simulink model "nms_sim_2D_cost"  (R2024b)
settings: Solver=ode15s  StartTime=0.0  StopTime=t_sim  MaxStep=dt_max  EnableMultiTasking=on
values from neighbouring files (symbols this model uses):
  a_BFSH = param_ctrl(35)*1    [setCtrlPar_optim_CPGreflex2001_2D.m]
  a_GAS = param_ctrl(37)*1    [setCtrlPar_optim_CPGreflex2001_2D.m]
  a_GLU = param_ctrl(31)*1    [setCtrlPar_optim_CPGreflex2001_2D.m]
  a_HAM = param_ctrl(33)*1    [setCtrlPar_optim_CPGreflex2001_2D.m]
  a_HFL = param_ctrl(32)*1    [setCtrlPar_optim_CPGreflex2001_2D.m]
  a_RF = param_ctrl(34)*1    [setCtrlPar_optim_CPGreflex2001_2D.m]
  a_SOL = param_ctrl(38)*1    [setCtrlPar_optim_CPGreflex2001_2D.m]
  a_TA = param_ctrl(39)*1    [setCtrlPar_optim_CPGreflex2001_2D.m]
  a_VAS = param_ctrl(36)*1    [setCtrlPar_optim_CPGreflex2001_2D.m]
  ai = param_ctrl(96)*2.0    [setCtrlPar_optim_CPGreflex2001_2D.m]
  b_BFSH = param_ctrl(52)*.51    [setCtrlPar_optim_CPGreflex2001_2D.m]
  b_BFSHGAS = param_ctrl(55)*.51    [setCtrlPar_optim_CPGreflex2001_2D.m]
  b_BFSHHAM = param_ctrl(54)*.51    [setCtrlPar_optim_CPGreflex2001_2D.m]
  b_BFSHVAS = param_ctrl(53)*.51    [setCtrlPar_optim_CPGreflex2001_2D.m]
  b_GAS = param_ctrl(59)*.51    [setCtrlPar_optim_CPGreflex2001_2D.m]
  b_GASBFSH = param_ctrl(60)*.51    [setCtrlPar_optim_CPGreflex2001_2D.m]
  b_GASSOL = param_ctrl(61)*.51    [setCtrlPar_optim_CPGreflex2001_2D.m]
  b_GLU = param_ctrl(40)*.51    [setCtrlPar_optim_CPGreflex2001_2D.m]
  b_GLUHAM = param_ctrl(42)*.51    [setCtrlPar_optim_CPGreflex2001_2D.m]
  b_GLUHFL = param_ctrl(41)*.51    [setCtrlPar_optim_CPGreflex2001_2D.m]
  b_HAM = param_ctrl(46)*.51    [setCtrlPar_optim_CPGreflex2001_2D.m]
  b_HAMBFSH = param_ctrl(48)*.51    [setCtrlPar_optim_CPGreflex2001_2D.m]
  b_HAMGLU = param_ctrl(47)*.51    [setCtrlPar_optim_CPGreflex2001_2D.m]
  b_HFL = param_ctrl(43)*.51    [setCtrlPar_optim_CPGreflex2001_2D.m]
  b_HFLGLU = param_ctrl(44)*.51    [setCtrlPar_optim_CPGreflex2001_2D.m]
  b_HFLRF = param_ctrl(45)*.51    [setCtrlPar_optim_CPGreflex2001_2D.m]
  b_RF = param_ctrl(49)*.51    [setCtrlPar_optim_CPGreflex2001_2D.m]
  b_RFHFL = param_ctrl(50)*.51    [setCtrlPar_optim_CPGreflex2001_2D.m]
  b_RFVAS = param_ctrl(51)*.51    [setCtrlPar_optim_CPGreflex2001_2D.m]
  b_SOL = param_ctrl(62)*.51    [setCtrlPar_optim_CPGreflex2001_2D.m]
  b_SOLGAS = param_ctrl(64)*.51    [setCtrlPar_optim_CPGreflex2001_2D.m]
  b_SOLTA = param_ctrl(63)*.51    [setCtrlPar_optim_CPGreflex2001_2D.m]
  b_TA = param_ctrl(65)*.51    [setCtrlPar_optim_CPGreflex2001_2D.m]
  b_TASOL = param_ctrl(66)*.51    [setCtrlPar_optim_CPGreflex2001_2D.m]
  b_VAS = param_ctrl(56)*.51    [setCtrlPar_optim_CPGreflex2001_2D.m]
  b_VASBFSH = param_ctrl(57)*.51    [setCtrlPar_optim_CPGreflex2001_2D.m]
  b_VASRF = param_ctrl(58)*.51    [setCtrlPar_optim_CPGreflex2001_2D.m]
  bias = param_ctrl(97)*2.5    [setCtrlPar_optim_CPGreflex2001_2D.m]
  c = 0.05    [nms_MS_2D_scaled.m]
  c_jointstop = 0.3 / (pi/180)    (= 17.1887338539)    [nms_MS_2D_scaled.m]
  D12_F = 0.16    *scaleL_JPhys    [nms_MechInit_2D_scaleSkel.m]
  D12_S = 0.2460	*sub_height    [nms_MechInit_2D_scaleSkel.m]
  D12_T = 0.2450  *sub_height    [nms_MechInit_2D_scaleSkel.m]
  D12y_F = 0.039  *sub_height    [nms_MechInit_2D_scaleSkel.m]
  D12z_HAT = 0.1    [nms_MS_2D_scaled.m]
  D13_F = 0.20    *scaleL_JPhys    [nms_MechInit_2D_scaleSkel.m]
  D1G_F = 0.14    *scaleL_JPhys    [nms_MechInit_2D_scaleSkel.m]
  D1G_HAT = 0.35  *scaleL_JPhys    [nms_MechInit_2D_scaleSkel.m]
  D1G_S = (0.3 - D12y_F/4)	*scaleL_JPhys    [nms_MechInit_2D_scaleSkel.m]
  D1G_T = (0.3 - D12y_F/4)	*scaleL_JPhys    [nms_MechInit_2D_scaleSkel.m]
  D1Gy_F = D12y_F*D1G_F/D12_F    (= 0.07)    [nms_MechInit_2D_scaleSkel.m]
  d_BFSH = param_ctrl(26)*1    [setCtrlPar_optim_CPGreflex2001_2D.m]
  d_GAS = param_ctrl(28)*1    [setCtrlPar_optim_CPGreflex2001_2D.m]
  d_GLU = param_ctrl(22)*1    [setCtrlPar_optim_CPGreflex2001_2D.m]
  d_HAM = param_ctrl(24)*1    [setCtrlPar_optim_CPGreflex2001_2D.m]
  d_HFL = param_ctrl(23)*1    [setCtrlPar_optim_CPGreflex2001_2D.m]
  d_RF = param_ctrl(25)*1    [setCtrlPar_optim_CPGreflex2001_2D.m]
  d_SOL = param_ctrl(29)*1    [setCtrlPar_optim_CPGreflex2001_2D.m]
  d_TA = param_ctrl(30)*1    [setCtrlPar_optim_CPGreflex2001_2D.m]
  d_VAS = param_ctrl(27)*1    [setCtrlPar_optim_CPGreflex2001_2D.m]
  DeltaThRef = 5e-3    (= 0.005)    [nms_MS_2D_scaled.m]
  dloptBFSH = 3.0    (= 3)    [setCtrlPar_optim_CPGreflex2001_2D.m]
  dloptGAS = 3.0    (= 3)    [setCtrlPar_optim_CPGreflex2001_2D.m]
  dloptGLU = 3.0    (= 3)    [setCtrlPar_optim_CPGreflex2001_2D.m]
  dloptHAM = 3.0    (= 3)    [setCtrlPar_optim_CPGreflex2001_2D.m]
  dloptHFL = 3.0    (= 3)    [setCtrlPar_optim_CPGreflex2001_2D.m]
  dloptRF = 3.0    (= 3)    [setCtrlPar_optim_CPGreflex2001_2D.m]
  dloptSOL = 3.0    (= 3)    [setCtrlPar_optim_CPGreflex2001_2D.m]
  dloptTA = 3.0    (= 3)    [setCtrlPar_optim_CPGreflex2001_2D.m]
  dloptVAS = 3.0    (= 3)    [setCtrlPar_optim_CPGreflex2001_2D.m]
  ec_BFSH = param_ctrl(80)*0.15    [setCtrlPar_optim_CPGreflex2001_2D.m]
  ec_GAS = param_ctrl(82)*0.15    [setCtrlPar_optim_CPGreflex2001_2D.m]
  ec_GLU = param_ctrl(76)*0.15    [setCtrlPar_optim_CPGreflex2001_2D.m]
  ec_HAM = param_ctrl(78)*0.15    [setCtrlPar_optim_CPGreflex2001_2D.m]
  ec_HFL = param_ctrl(77)*0.15    [setCtrlPar_optim_CPGreflex2001_2D.m]
  ec_RF = param_ctrl(79)*0.15    [setCtrlPar_optim_CPGreflex2001_2D.m]
  ec_TA = param_ctrl(84)*0.15    [setCtrlPar_optim_CPGreflex2001_2D.m]
  ec_VAS = param_ctrl(81)*0.15    [setCtrlPar_optim_CPGreflex2001_2D.m]
  eref = 0.04    [nms_MS_2D_scaled.m]
  eref_GAS = 0.1    [nms_MS_2D_scaled.m]
  eref_SOL = 0.1    [nms_MS_2D_scaled.m]
  es_BFSH = param_ctrl(89)*0.15    [setCtrlPar_optim_CPGreflex2001_2D.m]
  es_GAS = param_ctrl(91)*0.15    [setCtrlPar_optim_CPGreflex2001_2D.m]
  es_GLU = param_ctrl(85)*0.15    [setCtrlPar_optim_CPGreflex2001_2D.m]
  es_HAM = param_ctrl(87)*0.15    [setCtrlPar_optim_CPGreflex2001_2D.m]
  es_HFL = param_ctrl(86)*0.15    [setCtrlPar_optim_CPGreflex2001_2D.m]
  es_RF = param_ctrl(88)*0.15    [setCtrlPar_optim_CPGreflex2001_2D.m]
  es_TA = param_ctrl(93)*0.15    [setCtrlPar_optim_CPGreflex2001_2D.m]
  es_VAS = param_ctrl(90)*0.15    [setCtrlPar_optim_CPGreflex2001_2D.m]
  FmaxBFSH = 350    [nms_MS_2D_scaled.m]
  FmaxGAS = 2000    [nms_MS_2D_scaled.m]
  FmaxGLU = 4000    [nms_MS_2D_scaled.m]
  FmaxHAM = 2000    [nms_MS_2D_scaled.m]
  FmaxHFL = 2000    [nms_MS_2D_scaled.m]
  FmaxRF = 850    [nms_MS_2D_scaled.m]
  FmaxSOL = 4000    [nms_MS_2D_scaled.m]
  FmaxTA = 800    [nms_MS_2D_scaled.m]
  FmaxVAS = 5000    [nms_MS_2D_scaled.m]
  g = 9.81    [nms_MS_2D_scaled.m]
  gamma_4 = param_ctrl(11) * 1.7    [setCtrlPar_optim_CPGreflexsynergy2023_2D.m]
  h_BFSH = param_ctrl(71)*.1    [setCtrlPar_optim_CPGreflex2001_2D.m]
  h_GAS = param_ctrl(73)*.1    [setCtrlPar_optim_CPGreflex2001_2D.m]
  h_GLU = param_ctrl(67)*.1    [setCtrlPar_optim_CPGreflex2001_2D.m]
  h_HAM = param_ctrl(69)*.1    [setCtrlPar_optim_CPGreflex2001_2D.m]
  h_HFL = param_ctrl(68)*.1    [setCtrlPar_optim_CPGreflex2001_2D.m]
  h_RF = param_ctrl(70)*.1    [setCtrlPar_optim_CPGreflex2001_2D.m]
  h_SOL = param_ctrl(74)*.1    [setCtrlPar_optim_CPGreflex2001_2D.m]
  h_TA = param_ctrl(75)*.1    [setCtrlPar_optim_CPGreflex2001_2D.m]
  h_VAS = param_ctrl(72)*.1    [setCtrlPar_optim_CPGreflex2001_2D.m]
  HLCtrlPar = [theta_tgt l_clr alpha_tgt alpha_cd alpha_cv]    [setCtrlPar_optim_reflex2015_2D.m]
  In_F = 0.005    *scaleM*scaleL_JPhys^2    [nms_MechInit_2D_scaleSkel.m]
  In_HAT = 2.5    *scaleM*scaleL_JPhys^2    [nms_MechInit_2D_scaleSkel.m]
  In_S = 0.05     *scaleM*scaleL_JPhys^2    [nms_MechInit_2D_scaleSkel.m]
  In_T = 0.15     *scaleM*scaleL_JPhys^2    [nms_MechInit_2D_scaleSkel.m]
  init_exc = 0.01    [setInitPar_optim_2D.m]
  init_fm = 0.01    [setInitPar_optim_2D.m]
  init_lce = 1    [setInitPar_optim_2D.m]
  init_LCPG = param_ctrl(12) * 0.01    [setCtrlPar_optim_CPGreflexsynergy2023_2D.m]
  init_LStance = 1    [setInitPar_optim_2D.m]
  init_N1 = osc_signal1(phi_off_osc_ind)    [setCtrlPar_optim_CPGreflex2001_2D.m]
  ... (+441 more)
undefined symbols (not defined in the file or in its folder): cost_act_exponent, cost_v_tgt, flag_controller, Newton, nStep_obj, nStep_startKin, Raphson, sgn, SSW_kin, terrain_slope_angle, v_plateS1, X, Y, Z
libraries: nesl_utility x94, sm_lib x90, simulink x28, simulink_extras x12
(part 13 of 20)

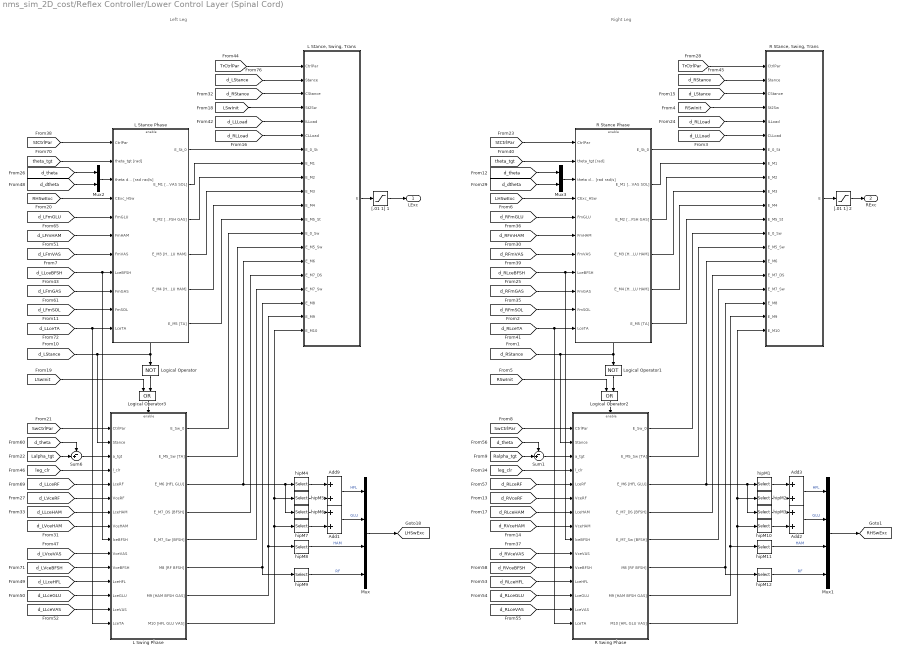
== system nms_sim_2D_cost/Reflex Controller/Lower Control Layer (Spinal Cord) ==
  note: Right Leg
  note: Left Leg
  Add{1..3,9} (4 alike) : Sum  Inputs=2
  L Stance Phase : Subsystem  TreatAsAtomicUnit=on
  "L Stance, Swing, Trans" : Subsystem
  L Swing Phase : Subsystem  TreatAsAtomicUnit=on
  Logical Operator : Logic  Operator=NOT  AllPortsSameDT=off  OutDataTypeStr=boolean
  Logical Operator1 : Logic  Operator=NOT  AllPortsSameDT=off  OutDataTypeStr=boolean
  Logical Operator2 : Logic  Operator=OR  AllPortsSameDT=off  OutDataTypeStr=boolean
  Logical Operator3 : Logic  Operator=OR  AllPortsSameDT=off  OutDataTypeStr=boolean
  Mux : Mux
  Mux1 : Mux
  Mux2 : Mux  Inputs=2
  Mux3 : Mux  Inputs=2
  R Stance Phase : Subsystem  TreatAsAtomicUnit=on
  "R Stance, Swing, Trans" : Subsystem
  R Swing Phase : Subsystem  TreatAsAtomicUnit=on
  Sum1 : Sum  Inputs=-+|
  Sum6 : Sum  Inputs=-+|
  "[.01 1] 1" : Saturate  UpperLimit=1  LowerLimit=0.01  ZeroCross=off
  "[.01 1] 2" : Saturate  UpperLimit=1  LowerLimit=0.01  ZeroCross=off
  hipM{1,4,9,12} (4 alike) : Selector  InputPortWidth=2  IndexOptions=Index vector (dialog)  Indices=1  OutputSizes=1
  hipM10 : Selector  InputPortWidth=3  IndexOptions=Index vector (dialog)  Indices=2  OutputSizes=1
  hipM{2,5,8,11} (4 alike) : Selector  InputPortWidth=3  IndexOptions=Index vector (dialog)  Indices=1  OutputSizes=1
  hipM3 : Selector  InputPortWidth=2  IndexOptions=Index vector (dialog)  Indices=2  OutputSizes=1
  hipM6 : Selector  InputPortWidth=2  IndexOptions=Index vector (dialog)  Indices=2  OutputSizes=1
  hipM7 : Selector  InputPortWidth=3  IndexOptions=Index vector (dialog)  Indices=2  OutputSizes=1
  LExc : Outport
  RExc : Outport  Port=2
  tag scope: LHSwExc=global, RHSwExc=global
  wires:
  L Stance Phase/4(E_M3 [HFL GLU HAM]) -> "L Stance, Swing, Trans"/10(E_M3)
  [StCtrlPar] -> L Stance Phase/1(CtrlPar)
  [theta_tgt] -> L Stance Phase/2(theta_tgt [rad])
  L Stance Phase/1(E_St_0) -> "L Stance, Swing, Trans"/7(E_0_St)
  L Stance Phase/2(E_M1 [GLU VAS SOL]) -> "L Stance, Swing, Trans"/8(E_M1)
  L Stance Phase/3(E_M2 [HAM VAS BFSH GAS]) -> "L Stance, Swing, Trans"/9(E_M2)
  Mux2/1 -> L Stance Phase/3(theta dtheta [rad rad/s])
  [d_LFmGAS] -> L Stance Phase/9(FmGAS)
  [d_LLLoad] -> "L Stance, Swing, Trans"/5(ILLoad)
  [d_LLceBFSH] -> L Swing Phase/9(lceBFSH), L Stance Phase/8(LceBFSH)
  [d_LFmGLU] -> L Stance Phase/5(FmGLU)
  [d_dtheta] -> Mux2/2
  [d_LFmHAM] -> L Stance Phase/6(FmHAM)
  [d_theta] -> Mux2/1
  [d_LFmVAS] -> L Stance Phase/7(FmVAS)
  [d_LFmSOL] -> L Stance Phase/10(FmSOL)
  "L Stance, Swing, Trans"/1(E) -> "[.01 1] 1"/1
  [d_RLLoad] -> "L Stance, Swing, Trans"/6(CLLoad)
  [LSwInit] -> "L Stance, Swing, Trans"/4(St2Sw)
  [TrCtrlPar] -> "L Stance, Swing, Trans"/1(CtrlPar)
  [d_LStance] -> "L Stance, Swing, Trans"/2(Stance)
  [d_RStance] -> "L Stance, Swing, Trans"/3(CStance)
  L Stance Phase/5(E_M4 [HFL GLU HAM]) -> "L Stance, Swing, Trans"/11(E_M4)
  L Stance Phase/6(E_M5 [TA]) -> "L Stance, Swing, Trans"/12(E_M5_St)
  L Swing Phase/1(E_Sw_0) -> "L Stance, Swing, Trans"/13(E_0_Sw)
  L Swing Phase/2(E_M5_Sw [TA]) -> "L Stance, Swing, Trans"/14(E_M5_Sw)
  L Swing Phase/3(E_M6 [HFL GLU]) -> hipM6/1, hipM4/1, "L Stance, Swing, Trans"/15(E_M6)
  L Swing Phase/5(E_M7_Sw [BFSH]) -> "L Stance, Swing, Trans"/17(E_M7_Sw)
  L Swing Phase/7(M9 [HAM BFSH GAS]) -> hipM8/1, "L Stance, Swing, Trans"/19(E_M9)
  Logical Operator/1 -> Logical Operator3/2
  [d_LStance] -> L Swing Phase/2(Stance), Logical Operator/1, L Stance Phase/Enable
  Logical Operator3/1 -> L Swing Phase/Enable
  [LSwInit] -> Logical Operator3/1
  [RHSwExc] -> L Stance Phase/4(CExc_HSw)
  [d_LLceTA] -> L Swing Phase/15(LceTA), L Stance Phase/11(LceTA)
  [SwCtrlPar] -> L Swing Phase/1(CtrlPar)
  [Lalpha_tgt] -> Sum6/2
  [d_theta] -> Sum6/1
  Sum6/1 -> L Swing Phase/3(a_tgt)
  [d_LLceRF] -> L Swing Phase/5(LceRF)
  [d_LVceRF] -> L Swing Phase/6(VceRF)
  [d_LLceHAM] -> L Swing Phase/7(LceHAM)
  [d_LVceHAM] -> L Swing Phase/8(VceHAM)
  Mux/1 -> [LHSwExc]
  R Stance Phase/6(E_M5 [TA]) -> "R Stance, Swing, Trans"/12(E_M5_St)
  R Stance Phase/5(E_M4 [HFL GLU HAM]) -> "R Stance, Swing, Trans"/11(E_M4)
  [RSwInit] -> Logical Operator2/1
  [LHSwExc] -> R Stance Phase/4(CExc_HSw)
  Logical Operator1/1 -> Logical Operator2/2
  [d_RFmGLU] -> R Stance Phase/5(FmGLU)
  [TrCtrlPar] -> "R Stance, Swing, Trans"/1(CtrlPar)
  [theta_tgt] -> R Stance Phase/2(theta_tgt [rad])
  [d_theta] -> Mux3/1
  [d_RFmHAM] -> R Stance Phase/6(FmHAM)
  [StCtrlPar] -> R Stance Phase/1(CtrlPar)
  [d_RFmVAS] -> R Stance Phase/7(FmVAS)
  [d_LStance] -> "R Stance, Swing, Trans"/3(CStance)
  [d_RStance] -> "R Stance, Swing, Trans"/2(Stance)
  [d_RFmSOL] -> R Stance Phase/10(FmSOL)
  Mux3/1 -> R Stance Phase/3(theta dtheta [rad rad/s])
  "R Stance, Swing, Trans"/1(E) -> "[.01 1] 2"/1
  [d_dtheta] -> Mux3/2
  R Stance Phase/1(E_St_0) -> "R Stance, Swing, Trans"/7(E_0_St)
  [RSwInit] -> "R Stance, Swing, Trans"/4(St2Sw)
  Logical Operator2/1 -> R Swing Phase/Enable
  [d_LLLoad] -> "R Stance, Swing, Trans"/6(CLLoad)
  R Swing Phase/7(M9 [HAM BFSH GAS]) -> "R Stance, Swing, Trans"/19(E_M9), hipM11/1
  [d_RFmGAS] -> R Stance Phase/9(FmGAS)
  R Stance Phase/3(E_M2 [HAM VAS BFSH GAS]) -> "R Stance, Swing, Trans"/9(E_M2)
  [d_RLLoad] -> "R Stance, Swing, Trans"/5(ILLoad)
  R Stance Phase/2(E_M1 [GLU VAS SOL]) -> "R Stance, Swing, Trans"/8(E_M1)
  R Swing Phase/5(E_M7_Sw [BFSH]) -> "R Stance, Swing, Trans"/17(E_M7_Sw)
  R Stance Phase/4(E_M3 [HFL GLU HAM]) -> "R Stance, Swing, Trans"/10(E_M3)
  [leg_clr] -> L Swing Phase/4(l_clr)
  [d_LLceVAS] -> L Swing Phase/14(LceVAS)
  [d_LVceBFSH] -> L Swing Phase/11(VceBFSH)
  [d_LLceHFL] -> L Swing Phase/12(LceHFL)
  [d_LVceVAS] -> L Swing Phase/10(VceVAS)
  [d_LLceGLU] -> L Swing Phase/13(LceGLU)
  L Swing Phase/4(E_M7_DS [BFSH]) -> "L Stance, Swing, Trans"/16(E_M7_DS)
  L Swing Phase/6(M8 [RF BFSH]) -> "L Stance, Swing, Trans"/18(E_M8), hipM9/1
  L Swing Phase/8(M10 [HFL GLU VAS]) -> hipM7/1, hipM5/1, "L Stance, Swing, Trans"/20(E_M10)
  Add9/1 -> Mux/1  "HFL"
  Add1/1 -> Mux/2  "GLU"
  hipM4/1 -> Add9/1
  hipM5/1 -> Add9/2
  hipM7/1 -> Add1/2
  hipM9/1 -> Mux/4  "RF"
  hipM8/1 -> Mux/3  "HAM"
  hipM6/1 -> Add1/1
  hipM1/1 -> Add3/1
  R Swing Phase/8(M10 [HFL GLU VAS]) -> hipM10/1, "R Stance, Swing, Trans"/20(E_M10), hipM2/1
  hipM10/1 -> Add2/2
  hipM12/1 -> Mux1/4  "RF"
  [d_RVceVAS] -> R Swing Phase/10(VceVAS)
  [d_RLceVAS] -> R Swing Phase/14(LceVAS)
  R Swing Phase/1(E_Sw_0) -> "R Stance, Swing, Trans"/13(E_0_Sw)
  hipM3/1 -> Add2/1
  [d_RLceHFL] -> R Swing Phase/12(LceHFL)
  [d_RLceGLU] -> R Swing Phase/13(LceGLU)
  R Swing Phase/3(E_M6 [HFL GLU]) -> "R Stance, Swing, Trans"/15(E_M6), hipM3/1, hipM1/1
  [d_RVceBFSH] -> R Swing Phase/11(VceBFSH)
  R Swing Phase/6(M8 [RF BFSH]) -> "R Stance, Swing, Trans"/18(E_M8), hipM12/1
  [leg_clr] -> R Swing Phase/4(l_clr)
  Add3/1 -> Mux1/1  "HFL"
  [SwCtrlPar] -> R Swing Phase/1(CtrlPar)
  hipM2/1 -> Add3/2
  [d_RLceTA] -> R Swing Phase/15(LceTA), R Stance Phase/11(LceTA)
  [d_RVceRF] -> R Swing Phase/6(VceRF)
  R Swing Phase/4(E_M7_DS [BFSH]) -> "R Stance, Swing, Trans"/16(E_M7_DS)
  Sum1/1 -> R Swing Phase/3(a_tgt)
  [d_RVceHAM] -> R Swing Phase/8(VceHAM)
  R Swing Phase/2(E_M5_Sw [TA]) -> "R Stance, Swing, Trans"/14(E_M5_Sw)
  [d_RLceRF] -> R Swing Phase/5(LceRF)
  hipM11/1 -> Mux1/3  "HAM"
  [d_RLceHAM] -> R Swing Phase/7(LceHAM)
  Mux1/1 -> [RHSwExc]
  [Ralpha_tgt] -> Sum1/2
  [d_theta] -> Sum1/1
  [d_RStance] -> R Swing Phase/2(Stance), Logical Operator1/1, R Stance Phase/Enable
  [d_RLceBFSH] -> R Swing Phase/9(lceBFSH), R Stance Phase/8(LceBFSH)
  Add2/1 -> Mux1/2  "GLU"
  "[.01 1] 1"/1 -> LExc/1
  "[.01 1] 2"/1 -> RExc/1

== system nms_sim_2D_cost/Body Mechanics/LBall Contact/2D Contact ==
  RefPt [m m] : Inport
  nVec [m m] : Inport  Port=2
  pVec [m m] : Inport  Port=3
  vVec [m/s m/s] : Inport  Port=4
  Contact! : EnablePort  StatesWhenEnabling=reset  ZeroCross=off
  Friction Switch : Subsystem
  Kinetic Friction Model : Subsystem
  Logical Operator : Logic  Operator=NOT  AllPortsSameDT=off  OutDataTypeStr=boolean
  Static Friction Model : Subsystem
  Sum : Sum
  Sum1 : Sum
  FnVec [N N] : Outport  OutputWhenDisabled=reset  InitialOutput=[0 0]  VectorParamsAs1DForOutWhenUnconnected=off
      settings: AttributesFormatString=when disabled: %<OutputWhenDisabled>
  FtVec [N N] : Outport  Port=2  OutputWhenDisabled=reset  InitialOutput=[0 0]  VectorParamsAs1DForOutWhenUnconnected=off
      settings: AttributesFormatString=when disabled: %<OutputWhenDisabled>
  wires:
  pVec [m m]/1 -> Static Friction Model/1(pos [m]), Kinetic Friction Model/2(pos [m m])
  vVec [m/s m/s]/1 -> Kinetic Friction Model/1(vel [m/s m/s]), Static Friction Model/2(vel [m/s m/s])
  Kinetic Friction Model/2(posFP [m m]) -> Static Friction Model/4(posFP [m])
  Friction Switch/1(Stiction) -> Static Friction Model/Enable, Logical Operator/1
  Logical Operator/1 -> Kinetic Friction Model/Enable
  nVec [m m]/1 -> Kinetic Friction Model/4(nVec [m m])
  Kinetic Friction Model/4(Stiction!) -> Friction Switch/2(Stick!)
  Static Friction Model/1(F_n Stick [N N]) -> Sum1/1
  Kinetic Friction Model/6(F_n Slide [N N]) -> Sum1/2
  Kinetic Friction Model/5(F_t Slide [N N]) -> Sum/2
  Static Friction Model/2(F_t Stick [N N]) -> Sum/1
  Sum1/1 -> FnVec [N N]/1  "F_nVec"
  Sum/1 -> FtVec [N N]/1  "F_tVec"
  Static Friction Model/3(Sliding!) -> Friction Switch/1(Slide!)
  RefPt [m m]/1 -> Kinetic Friction Model/3(RefPt [m m])
  Kinetic Friction Model/3(nVec FP [m m]) -> Static Friction Model/5(nVecFP [m m])
  Kinetic Friction Model/1(RefPtFP [m m]) -> Static Friction Model/3(RefPtFP [m m])

== system nms_sim_2D_cost/Body Mechanics/LHeel Contact/2D Contact ==
  RefPt [m m] : Inport
  nVec [m m] : Inport  Port=2
  pVec [m m] : Inport  Port=3
  vVec [m/s m/s] : Inport  Port=4
  Contact! : EnablePort  StatesWhenEnabling=reset  ZeroCross=off
  Friction Switch : Subsystem
  Kinetic Friction Model : Subsystem
  Logical Operator : Logic  Operator=NOT  AllPortsSameDT=off  OutDataTypeStr=boolean
  Static Friction Model : Subsystem
  Sum : Sum
  Sum1 : Sum
  FnVec [N N] : Outport  OutputWhenDisabled=reset  InitialOutput=[0 0]  VectorParamsAs1DForOutWhenUnconnected=off
      settings: AttributesFormatString=when disabled: %<OutputWhenDisabled>
  FtVec [N N] : Outport  Port=2  OutputWhenDisabled=reset  InitialOutput=[0 0]  VectorParamsAs1DForOutWhenUnconnected=off
      settings: AttributesFormatString=when disabled: %<OutputWhenDisabled>
  wires:
  pVec [m m]/1 -> Static Friction Model/1(pos [m]), Kinetic Friction Model/2(pos [m m])
  vVec [m/s m/s]/1 -> Kinetic Friction Model/1(vel [m/s m/s]), Static Friction Model/2(vel [m/s m/s])
  Kinetic Friction Model/2(posFP [m m]) -> Static Friction Model/4(posFP [m])
  Friction Switch/1(Stiction) -> Static Friction Model/Enable, Logical Operator/1
  Logical Operator/1 -> Kinetic Friction Model/Enable
  nVec [m m]/1 -> Kinetic Friction Model/4(nVec [m m])
  Kinetic Friction Model/4(Stiction!) -> Friction Switch/2(Stick!)
  Static Friction Model/1(F_n Stick [N N]) -> Sum1/1
  Kinetic Friction Model/6(F_n Slide [N N]) -> Sum1/2
  Kinetic Friction Model/5(F_t Slide [N N]) -> Sum/2
  Static Friction Model/2(F_t Stick [N N]) -> Sum/1
  Sum1/1 -> FnVec [N N]/1  "F_nVec"
  Sum/1 -> FtVec [N N]/1  "F_tVec"
  Static Friction Model/3(Sliding!) -> Friction Switch/1(Slide!)
  RefPt [m m]/1 -> Kinetic Friction Model/3(RefPt [m m])
  Kinetic Friction Model/3(nVec FP [m m]) -> Static Friction Model/5(nVecFP [m m])
  Kinetic Friction Model/1(RefPtFP [m m]) -> Static Friction Model/3(RefPtFP [m m])

== system nms_sim_2D_cost/Body Mechanics/RBall Contact/2D Contact ==
  RefPt [m m] : Inport
  nVec [m m] : Inport  Port=2
  pVec [m m] : Inport  Port=3
  vVec [m/s m/s] : Inport  Port=4
  Contact! : EnablePort  StatesWhenEnabling=reset  ZeroCross=off
  Friction Switch : Subsystem
  Kinetic Friction Model : Subsystem
  Logical Operator : Logic  Operator=NOT  AllPortsSameDT=off  OutDataTypeStr=boolean
  Static Friction Model : Subsystem
  Sum : Sum
  Sum1 : Sum
  FnVec [N N] : Outport  OutputWhenDisabled=reset  InitialOutput=[0 0]  VectorParamsAs1DForOutWhenUnconnected=off
      settings: AttributesFormatString=when disabled: %<OutputWhenDisabled>
  FtVec [N N] : Outport  Port=2  OutputWhenDisabled=reset  InitialOutput=[0 0]  VectorParamsAs1DForOutWhenUnconnected=off
      settings: AttributesFormatString=when disabled: %<OutputWhenDisabled>
  wires:
  pVec [m m]/1 -> Static Friction Model/1(pos [m]), Kinetic Friction Model/2(pos [m m])
  vVec [m/s m/s]/1 -> Kinetic Friction Model/1(vel [m/s m/s]), Static Friction Model/2(vel [m/s m/s])
  Kinetic Friction Model/2(posFP [m m]) -> Static Friction Model/4(posFP [m])
  Friction Switch/1(Stiction) -> Static Friction Model/Enable, Logical Operator/1
  Logical Operator/1 -> Kinetic Friction Model/Enable
  nVec [m m]/1 -> Kinetic Friction Model/4(nVec [m m])
  Kinetic Friction Model/4(Stiction!) -> Friction Switch/2(Stick!)
  Static Friction Model/1(F_n Stick [N N]) -> Sum1/1
  Kinetic Friction Model/6(F_n Slide [N N]) -> Sum1/2
  Kinetic Friction Model/5(F_t Slide [N N]) -> Sum/2
  Static Friction Model/2(F_t Stick [N N]) -> Sum/1
  Sum1/1 -> FnVec [N N]/1  "F_nVec"
  Sum/1 -> FtVec [N N]/1  "F_tVec"
  Static Friction Model/3(Sliding!) -> Friction Switch/1(Slide!)
  RefPt [m m]/1 -> Kinetic Friction Model/3(RefPt [m m])
  Kinetic Friction Model/3(nVec FP [m m]) -> Static Friction Model/5(nVecFP [m m])
  Kinetic Friction Model/1(RefPtFP [m m]) -> Static Friction Model/3(RefPtFP [m m])

== system nms_sim_2D_cost/Body Mechanics/RHeel Contact/2D Contact ==
  RefPt [m m] : Inport
  nVec [m m] : Inport  Port=2
  pVec [m m] : Inport  Port=3
  vVec [m/s m/s] : Inport  Port=4
  Contact! : EnablePort  StatesWhenEnabling=reset  ZeroCross=off
  Friction Switch : Subsystem
  Kinetic Friction Model : Subsystem
  Logical Operator : Logic  Operator=NOT  AllPortsSameDT=off  OutDataTypeStr=boolean
  Static Friction Model : Subsystem
  Sum : Sum
  Sum1 : Sum
  FnVec [N N] : Outport  OutputWhenDisabled=reset  InitialOutput=[0 0]  VectorParamsAs1DForOutWhenUnconnected=off
      settings: AttributesFormatString=when disabled: %<OutputWhenDisabled>
  FtVec [N N] : Outport  Port=2  OutputWhenDisabled=reset  InitialOutput=[0 0]  VectorParamsAs1DForOutWhenUnconnected=off
      settings: AttributesFormatString=when disabled: %<OutputWhenDisabled>
  wires:
  pVec [m m]/1 -> Static Friction Model/1(pos [m]), Kinetic Friction Model/2(pos [m m])
  vVec [m/s m/s]/1 -> Kinetic Friction Model/1(vel [m/s m/s]), Static Friction Model/2(vel [m/s m/s])
  Kinetic Friction Model/2(posFP [m m]) -> Static Friction Model/4(posFP [m])
  Friction Switch/1(Stiction) -> Static Friction Model/Enable, Logical Operator/1
  Logical Operator/1 -> Kinetic Friction Model/Enable
  nVec [m m]/1 -> Kinetic Friction Model/4(nVec [m m])
  Kinetic Friction Model/4(Stiction!) -> Friction Switch/2(Stick!)
  Static Friction Model/1(F_n Stick [N N]) -> Sum1/1
  Kinetic Friction Model/6(F_n Slide [N N]) -> Sum1/2
  Kinetic Friction Model/5(F_t Slide [N N]) -> Sum/2
  Static Friction Model/2(F_t Stick [N N]) -> Sum/1
  Sum1/1 -> FnVec [N N]/1  "F_nVec"
  Sum/1 -> FtVec [N N]/1  "F_tVec"
  Static Friction Model/3(Sliding!) -> Friction Switch/1(Slide!)
  RefPt [m m]/1 -> Kinetic Friction Model/3(RefPt [m m])
  Kinetic Friction Model/3(nVec FP [m m]) -> Static Friction Model/5(nVecFP [m m])
  Kinetic Friction Model/1(RefPtFP [m m]) -> Static Friction Model/3(RefPtFP [m m])

== system nms_sim_2D_cost/CPG-reflex Controller/Alpha moto-neuron/sigmoid function ==
  u : Inport
  Fcn : Fcn  Expr=2/(1+exp(-0.25*u(1)))-1
  Max : MinMax  Function=max  Inputs=2
  Zero : Constant  Value=0  OutDataTypeStr=Inherit: Inherit via back propagation
  LExcGLU : Outport
  wires:
  u/1 -> Fcn/1
  Fcn/1 -> Max/1
  Max/1 -> LExcGLU/1
  Zero/1 -> Max/2

== system nms_sim_2D_cost/CPG-reflex Controller/Alpha moto-neuron1/sigmoid function ==
  u : Inport
  Fcn : Fcn  Expr=2/(1+exp(-0.25*u(1)))-1
  Max : MinMax  Function=max  Inputs=2
  Zero : Constant  Value=0  OutDataTypeStr=Inherit: Inherit via back propagation
  LExcHAM : Outport
  wires:
  u/1 -> Fcn/1
  Fcn/1 -> Max/1
  Max/1 -> LExcHAM/1
  Zero/1 -> Max/2

== system nms_sim_2D_cost/CPG-reflex Controller/Alpha moto-neuron18/sigmoid function ==
  u : Inport
  Fcn : Fcn  Expr=2/(1+exp(-0.25*u(1)))-1
  Max : MinMax  Function=max  Inputs=2
  Zero : Constant  Value=0  OutDataTypeStr=Inherit: Inherit via back propagation
  RExc : Outport
  wires:
  u/1 -> Fcn/1
  Fcn/1 -> Max/1
  Max/1 -> RExc/1
  Zero/1 -> Max/2

== system nms_sim_2D_cost/CPG-reflex Controller/Alpha moto-neuron19/sigmoid function ==
  u : Inport
  Fcn : Fcn  Expr=2/(1+exp(-0.25*u(1)))-1
  Max : MinMax  Function=max  Inputs=2
  Zero : Constant  Value=0  OutDataTypeStr=Inherit: Inherit via back propagation
  RExc : Outport
  wires:
  u/1 -> Fcn/1
  Fcn/1 -> Max/1
  Max/1 -> RExc/1
  Zero/1 -> Max/2

== system nms_sim_2D_cost/CPG-reflex Controller/Alpha moto-neuron2/sigmoid function ==
  u : Inport
  Fcn : Fcn  Expr=2/(1+exp(-0.25*u(1)))-1
  Max : MinMax  Function=max  Inputs=2
  Zero : Constant  Value=0  OutDataTypeStr=Inherit: Inherit via back propagation
  LExc : Outport
  wires:
  u/1 -> Fcn/1
  Fcn/1 -> Max/1
  Max/1 -> LExc/1
  Zero/1 -> Max/2

== system nms_sim_2D_cost/CPG-reflex Controller/Alpha moto-neuron20/sigmoid function ==
  u : Inport
  Fcn : Fcn  Expr=2/(1+exp(-0.25*u(1)))-1
  Max : MinMax  Function=max  Inputs=2
  Zero : Constant  Value=0  OutDataTypeStr=Inherit: Inherit via back propagation
  RExc : Outport
  wires:
  u/1 -> Fcn/1
  Fcn/1 -> Max/1
  Max/1 -> RExc/1
  Zero/1 -> Max/2

== system nms_sim_2D_cost/CPG-reflex Controller/Alpha moto-neuron21/sigmoid function ==
  u : Inport
  Fcn : Fcn  Expr=2/(1+exp(-0.25*u(1)))-1
  Max : MinMax  Function=max  Inputs=2
  Zero : Constant  Value=0  OutDataTypeStr=Inherit: Inherit via back propagation
  RExc : Outport
  wires:
  u/1 -> Fcn/1
  Fcn/1 -> Max/1
  Max/1 -> RExc/1
  Zero/1 -> Max/2

== system nms_sim_2D_cost/CPG-reflex Controller/Alpha moto-neuron22/sigmoid function ==
  u : Inport
  Fcn : Fcn  Expr=2/(1+exp(-0.25*u(1)))-1
  Max : MinMax  Function=max  Inputs=2
  Zero : Constant  Value=0  OutDataTypeStr=Inherit: Inherit via back propagation
  RExc : Outport
  wires:
  u/1 -> Fcn/1
  Fcn/1 -> Max/1
  Max/1 -> RExc/1
  Zero/1 -> Max/2

== system nms_sim_2D_cost/CPG-reflex Controller/Alpha moto-neuron23/sigmoid function ==
  u : Inport
  Fcn : Fcn  Expr=2/(1+exp(-0.25*u(1)))-1
  Max : MinMax  Function=max  Inputs=2
  Zero : Constant  Value=0  OutDataTypeStr=Inherit: Inherit via back propagation
  RExc : Outport
  wires:
  u/1 -> Fcn/1
  Fcn/1 -> Max/1
  Max/1 -> RExc/1
  Zero/1 -> Max/2

== system nms_sim_2D_cost/CPG-reflex Controller/Alpha moto-neuron24/sigmoid function ==
  u : Inport
  Fcn : Fcn  Expr=2/(1+exp(-0.25*u(1)))-1
  Max : MinMax  Function=max  Inputs=2
  Zero : Constant  Value=0  OutDataTypeStr=Inherit: Inherit via back propagation
  RExc : Outport
  wires:
  u/1 -> Fcn/1
  Fcn/1 -> Max/1
  Max/1 -> RExc/1
  Zero/1 -> Max/2

== system nms_sim_2D_cost/CPG-reflex Controller/Alpha moto-neuron25/sigmoid function ==
  u : Inport
  Fcn : Fcn  Expr=2/(1+exp(-0.25*u(1)))-1
  Max : MinMax  Function=max  Inputs=2
  Zero : Constant  Value=0  OutDataTypeStr=Inherit: Inherit via back propagation
  RExc : Outport
  wires:
  u/1 -> Fcn/1
  Fcn/1 -> Max/1
  Max/1 -> RExc/1
  Zero/1 -> Max/2

== system nms_sim_2D_cost/CPG-reflex Controller/Alpha moto-neuron26/sigmoid function ==
  u : Inport
  Fcn : Fcn  Expr=2/(1+exp(-0.25*u(1)))-1
  Max : MinMax  Function=max  Inputs=2
  Zero : Constant  Value=0  OutDataTypeStr=Inherit: Inherit via back propagation
  RExc : Outport
  wires:
  u/1 -> Fcn/1
  Fcn/1 -> Max/1
  Max/1 -> RExc/1
  Zero/1 -> Max/2

== system nms_sim_2D_cost/CPG-reflex Controller/Alpha moto-neuron3/sigmoid function ==
  u : Inport
  Fcn : Fcn  Expr=2/(1+exp(-0.25*u(1)))-1
  Max : MinMax  Function=max  Inputs=2
  Zero : Constant  Value=0  OutDataTypeStr=Inherit: Inherit via back propagation
  LExc : Outport
  wires:
  u/1 -> Fcn/1
  Fcn/1 -> Max/1
  Max/1 -> LExc/1
  Zero/1 -> Max/2

== system nms_sim_2D_cost/CPG-reflex Controller/Alpha moto-neuron4/sigmoid function ==
  u : Inport
  Fcn : Fcn  Expr=2/(1+exp(-0.25*u(1)))-1
  Max : MinMax  Function=max  Inputs=2
  Zero : Constant  Value=0  OutDataTypeStr=Inherit: Inherit via back propagation
  LExcBFSH : Outport
  wires:
  u/1 -> Fcn/1
  Fcn/1 -> Max/1
  Max/1 -> LExcBFSH/1
  Zero/1 -> Max/2

== system nms_sim_2D_cost/CPG-reflex Controller/Alpha moto-neuron5/sigmoid function ==
  u : Inport
  Fcn : Fcn  Expr=2/(1+exp(-0.25*u(1)))-1
  Max : MinMax  Function=max  Inputs=2
  Zero : Constant  Value=0  OutDataTypeStr=Inherit: Inherit via back propagation
  LExc : Outport
  wires:
  u/1 -> Fcn/1
  Fcn/1 -> Max/1
  Max/1 -> LExc/1
  Zero/1 -> Max/2

== system nms_sim_2D_cost/CPG-reflex Controller/Alpha moto-neuron6/sigmoid function ==
  u : Inport
  Fcn : Fcn  Expr=2/(1+exp(-0.25*u(1)))-1
  Max : MinMax  Function=max  Inputs=2
  Zero : Constant  Value=0  OutDataTypeStr=Inherit: Inherit via back propagation
  LExcSOL : Outport
  wires:
  u/1 -> Fcn/1
  Fcn/1 -> Max/1
  Max/1 -> LExcSOL/1
  Zero/1 -> Max/2

== system nms_sim_2D_cost/CPG-reflex Controller/Alpha moto-neuron7/sigmoid function ==
  u : Inport
  Fcn : Fcn  Expr=2/(1+exp(-0.25*u(1)))-1
  Max : MinMax  Function=max  Inputs=2
  Zero : Constant  Value=0  OutDataTypeStr=Inherit: Inherit via back propagation
  LExcTA : Outport
  wires:
  u/1 -> Fcn/1
  Fcn/1 -> Max/1
  Max/1 -> LExcTA/1
  Zero/1 -> Max/2

== system nms_sim_2D_cost/CPG-reflex Controller/Alpha moto-neuron8/sigmoid function ==
  u : Inport
  Fcn : Fcn  Expr=2/(1+exp(-0.25*u(1)))-1
  Max : MinMax  Function=max  Inputs=2
  Zero : Constant  Value=0  OutDataTypeStr=Inherit: Inherit via back propagation
  LExcBFSH : Outport
  wires:
  u/1 -> Fcn/1
  Fcn/1 -> Max/1
  Max/1 -> LExcBFSH/1
  Zero/1 -> Max/2

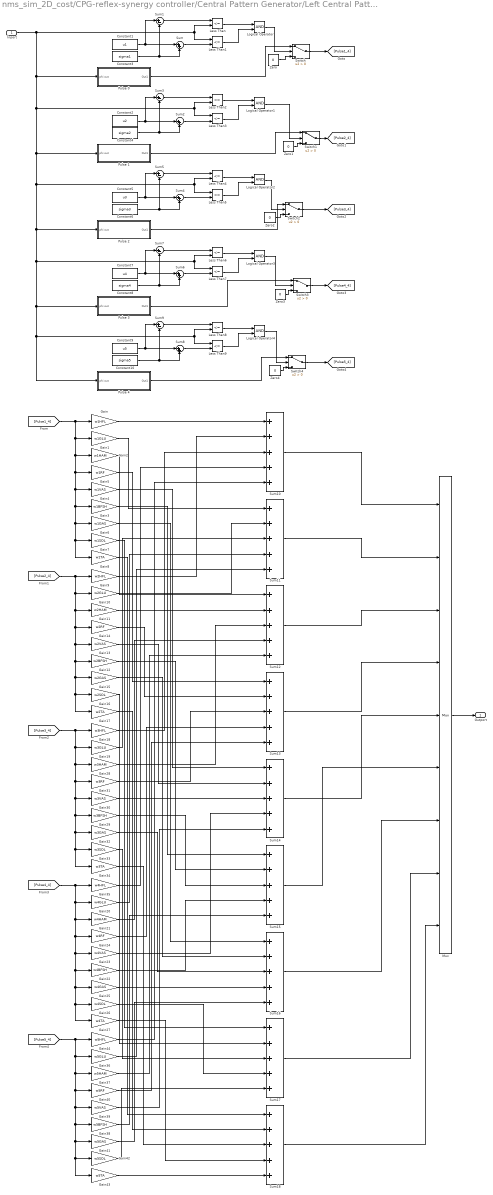
== system nms_sim_2D_cost/CPG-reflex-synergy controller/Central Pattern Generator/Left Central Pattern Generator ==
  Inport : Inport
  Constant1 : Constant  Value=u1
  Constant10 : Constant  Value=sigma5
  Constant2 : Constant  Value=u2
  Constant3 : Constant  Value=sigma1
  Constant4 : Constant  Value=sigma2
  Constant5 : Constant  Value=u3
  Constant6 : Constant  Value=sigma3
  Constant7 : Constant  Value=u4
  Constant8 : Constant  Value=sigma4
  Constant9 : Constant  Value=u5
  Gain : Gain  Gain=w1HFL
  Gain1 : Gain  Gain=w1GLU
  Gain10 : Gain  Gain=w2GLU
  Gain11 : Gain  Gain=w2HAM
  Gain12 : Gain  Gain=w2BFSH
  Gain13 : Gain  Gain=w2VAS
  Gain14 : Gain  Gain=w2RF
  Gain15 : Gain  Gain=w2GAS
  Gain16 : Gain  Gain=w2SOL
  Gain17 : Gain  Gain=w2TA
  Gain18 : Gain  Gain=w3HFL
  Gain19 : Gain  Gain=w3GLU
  Gain2 : Gain  Gain=w1HAM
  Gain20 : Gain  Gain=w4GLU
  Gain21 : Gain  Gain=w4HAM
  Gain22 : Gain  Gain=w4BFSH
  Gain23 : Gain  Gain=w4VAS
  Gain24 : Gain  Gain=w4RF
  Gain25 : Gain  Gain=w4GAS
  Gain26 : Gain  Gain=w4SOL
  Gain27 : Gain  Gain=w4TA
  Gain28 : Gain  Gain=w3HAM
  Gain29 : Gain  Gain=w3BFSH
  Gain3 : Gain  Gain=w1BFSH
  Gain30 : Gain  Gain=w3VAS
  Gain31 : Gain  Gain=w3RF
  Gain32 : Gain  Gain=w3GAS
  Gain33 : Gain  Gain=w3SOL
  Gain34 : Gain  Gain=w3TA
  Gain35 : Gain  Gain=w4HFL
  Gain36 : Gain  Gain=w5GLU
  Gain37 : Gain  Gain=w5HAM
  Gain38 : Gain  Gain=w5BFSH
  Gain39 : Gain  Gain=w5VAS
  Gain4 : Gain  Gain=w1VAS
  Gain40 : Gain  Gain=w5RF
  Gain41 : Gain  Gain=w5GAS
  Gain42 : Gain  Gain=w5SOL
  Gain43 : Gain  Gain=w5TA
  Gain44 : Gain  Gain=w5HFL
  Gain5 : Gain  Gain=w1RF
  Gain6 : Gain  Gain=w1GAS
  Gain7 : Gain  Gain=w1SOL
  Gain8 : Gain  Gain=w1TA
  Gain9 : Gain  Gain=w2HFL
  Less Than{,1..9} (10 alike) : RelationalOperator  Operator=<=  OutDataTypeStr=boolean  RndMeth=Simplest  InputSameDT=off
  Logical Operator{,1..4} (5 alike) : Logic  AllPortsSameDT=off  OutDataTypeStr=boolean
  Mux : Mux  Inputs=9
  Pulse 0 : Subsystem
  Pulse 1 : Subsystem
  Pulse 2 : Subsystem
  Pulse 3 : Subsystem
  Pulse 4 : Subsystem
  Sum{,2,4,6,8} (5 alike) : Sum  Inputs=|++
  Sum{1,3,5,7,9} (5 alike) : Sum  Inputs=|+-
  Sum{10..18} (9 alike) : Sum  Inputs=+++++
  Switch{,1..4} (5 alike) : Switch  Criteria=u2 > Threshold  SaturateOnIntegerOverflow=off  InputSameDT=off
  Zero{,1..4} (5 alike) : Constant  Value=0  OutDataTypeStr=Inherit: Inherit via back propagation
  Outport : Outport
  wires:
  Pulse 2/1(Out1) -> Switch2/1
  Pulse 4/1(Out1) -> Switch4/1
  Logical Operator2/1 -> Switch2/2
  Constant6/1 -> Sum5/2, Sum4/2
  Constant5/1 -> Sum5/1, Sum4/1
  Less Than5/1 -> Logical Operator2/2
  Less Than4/1 -> Logical Operator2/1
  Sum/1 -> Less Than1/2
  Pulse 0/1(Out1) -> Switch/1
  Constant3/1 -> Sum1/2, Sum/2
  Less Than/1 -> Logical Operator/1
  Zero4/1 -> Switch4/3
  Switch4/1 -> [Pulse5_4]
  Logical Operator/1 -> Switch/2
  Logical Operator1/1 -> Switch1/2
  Pulse 1/1(Out1) -> Switch1/1
  Sum1/1 -> Less Than/1
  Zero2/1 -> Switch2/3
  Switch2/1 -> [Pulse3_4]
  Pulse 3/1(Out1) -> Switch3/1
  Sum5/1 -> Less Than4/1
  Less Than2/1 -> Logical Operator1/1
  Switch/1 -> [Pulse1_4]
  Zero3/1 -> Switch3/3
  Switch3/1 -> [Pulse4_4]
  Sum3/1 -> Less Than2/1
  Constant7/1 -> Sum6/1, Sum7/1
  Constant4/1 -> Sum2/2, Sum3/2
  Sum6/1 -> Less Than7/2
  Constant8/1 -> Sum6/2, Sum7/2
  Logical Operator4/1 -> Switch4/2
  Sum9/1 -> Less Than8/1
  Zero/1 -> Switch/3
  Sum8/1 -> Less Than9/2
  Less Than1/1 -> Logical Operator/2
  Less Than6/1 -> Logical Operator3/1
  Switch1/1 -> [Pulse2_4]
  Constant10/1 -> Sum9/2, Sum8/2
  Less Than7/1 -> Logical Operator3/2
  Logical Operator3/1 -> Switch3/2
  Constant2/1 -> Sum2/1, Sum3/1
  Less Than8/1 -> Logical Operator4/1
  Zero1/1 -> Switch1/3
  Sum2/1 -> Less Than3/2
  Sum7/1 -> Less Than6/1
  Less Than9/1 -> Logical Operator4/2
  Sum4/1 -> Less Than5/2
  Less Than3/1 -> Logical Operator1/2
  Constant9/1 -> Sum9/1, Sum8/1
  Constant1/1 -> Sum1/1, Sum/1
  Inport/1 -> Less Than1/1, Less Than/2, Less Than5/1, Less Than4/2, Less Than9/1, Less Than8/2, Pulse 4/1(phi out), Pulse 3/1(phi out), Less Than6/2, Less Than7/1, Pulse 2/1(phi out), Pulse 1/1(phi out), Less Than2/2, Less Than3/1, Pulse 0/1(phi out)
  [Pulse1_4] -> Gain3/1, Gain8/1, Gain7/1, Gain6/1, Gain4/1, Gain5/1, Gain2/1, Gain1/1, Gain/1
  [Pulse2_4] -> Gain9/1, Gain10/1, Gain11/1, Gain14/1, Gain13/1, Gain15/1, Gain16/1, Gain17/1, Gain12/1
  [Pulse4_4] -> Gain22/1, Gain27/1, Gain26/1, Gain25/1, Gain23/1, Gain24/1, Gain21/1, Gain20/1, Gain35/1
  [Pulse3_4] -> Gain18/1, Gain19/1, Gain28/1, Gain31/1, Gain30/1, Gain32/1, Gain33/1, Gain34/1, Gain29/1
  [Pulse5_4] -> Gain44/1, Gain36/1, Gain37/1, Gain40/1, Gain39/1, Gain41/1, Gain42/1, Gain43/1, Gain38/1
  Gain/1 -> Sum10/1
  Gain9/1 -> Sum10/2
  Gain18/1 -> Sum10/3
  Gain35/1 -> Sum10/4
  Gain44/1 -> Sum10/5
  Gain43/1 -> Sum18/5
  Gain27/1 -> Sum18/4
  Gain34/1 -> Sum18/3
  Gain17/1 -> Sum18/2
  Gain8/1 -> Sum18/1
  Gain42/1 -> Sum17/5
  Gain26/1 -> Sum17/4
  Gain33/1 -> Sum17/3
  Gain16/1 -> Sum17/2
  Gain7/1 -> Sum17/1
  Gain1/1 -> Sum11/1
  Gain10/1 -> Sum11/2
  Gain19/1 -> Sum11/3
  Gain20/1 -> Sum11/4
  Gain36/1 -> Sum11/5
  Gain2/1 -> Sum12/1
  Gain11/1 -> Sum12/2
  Gain28/1 -> Sum12/3
  Gain21/1 -> Sum12/4
  Gain37/1 -> Sum12/5
  Gain31/1 -> Sum13/3
  Gain5/1 -> Sum13/1
  Gain14/1 -> Sum13/2
  Gain24/1 -> Sum13/4
  Gain40/1 -> Sum13/5
  Gain30/1 -> Sum14/3
  Gain23/1 -> Sum14/4
  Gain39/1 -> Sum14/5
  Gain38/1 -> Sum15/5
  Gain41/1 -> Sum16/5
  Gain25/1 -> Sum16/4
  Gain22/1 -> Sum15/4
  Gain32/1 -> Sum16/3
  Gain29/1 -> Sum15/3
  Gain15/1 -> Sum16/2
  Gain12/1 -> Sum15/2
  Gain13/1 -> Sum14/2
  Gain6/1 -> Sum16/1
  Gain3/1 -> Sum15/1
  Gain4/1 -> Sum14/1
  Sum10/1 -> Mux/1
  Sum11/1 -> Mux/2
  Sum12/1 -> Mux/3
  Sum13/1 -> Mux/4
  Sum14/1 -> Mux/5
  Sum15/1 -> Mux/6
  Sum16/1 -> Mux/7
  Sum17/1 -> Mux/8
  Sum18/1 -> Mux/9
  Mux/1 -> Outport/1

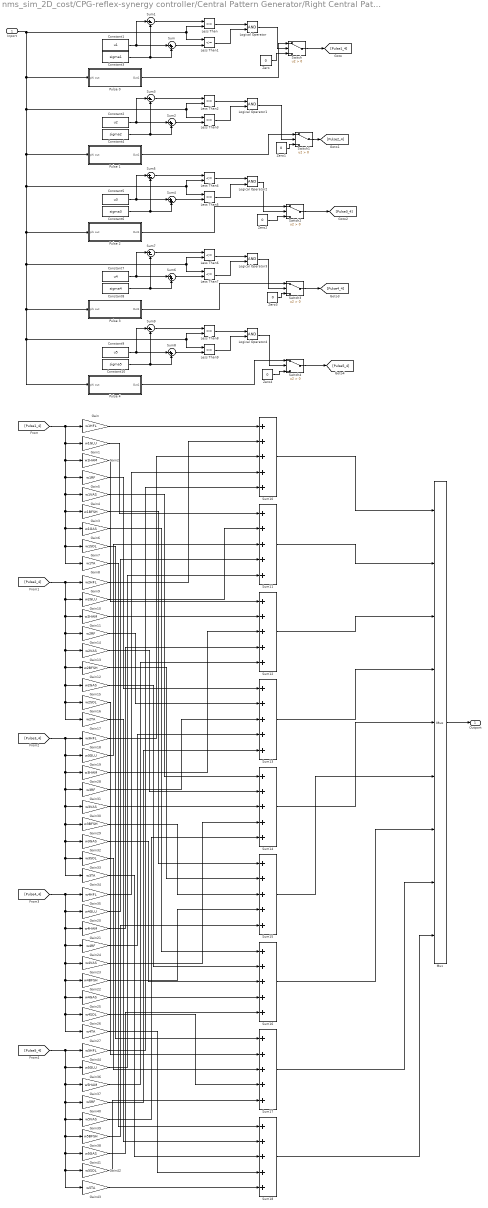
== system nms_sim_2D_cost/CPG-reflex-synergy controller/Central Pattern Generator/Right Central Pattern Generator ==
  Inport : Inport
  Constant1 : Constant  Value=u1
  Constant10 : Constant  Value=sigma5
  Constant2 : Constant  Value=u2
  Constant3 : Constant  Value=sigma1
  Constant4 : Constant  Value=sigma2
  Constant5 : Constant  Value=u3
  Constant6 : Constant  Value=sigma3
  Constant7 : Constant  Value=u4
  Constant8 : Constant  Value=sigma4
  Constant9 : Constant  Value=u5
  Gain : Gain  Gain=w1HFL
  Gain1 : Gain  Gain=w1GLU
  Gain10 : Gain  Gain=w2GLU
  Gain11 : Gain  Gain=w2HAM
  Gain12 : Gain  Gain=w2BFSH
  Gain13 : Gain  Gain=w2VAS
  Gain14 : Gain  Gain=w2RF
  Gain15 : Gain  Gain=w2GAS
  Gain16 : Gain  Gain=w2SOL
  Gain17 : Gain  Gain=w2TA
  Gain18 : Gain  Gain=w3HFL
  Gain19 : Gain  Gain=w3GLU
  Gain2 : Gain  Gain=w1HAM
  Gain20 : Gain  Gain=w4GLU
  Gain21 : Gain  Gain=w4HAM
  Gain22 : Gain  Gain=w4BFSH
  Gain23 : Gain  Gain=w4VAS
  Gain24 : Gain  Gain=w4RF
  Gain25 : Gain  Gain=w4GAS
  Gain26 : Gain  Gain=w4SOL
  Gain27 : Gain  Gain=w4TA
  Gain28 : Gain  Gain=w3HAM
  Gain29 : Gain  Gain=w3BFSH
  Gain3 : Gain  Gain=w1BFSH
  Gain30 : Gain  Gain=w3VAS
  Gain31 : Gain  Gain=w3RF
  Gain32 : Gain  Gain=w3GAS
  Gain33 : Gain  Gain=w3SOL
  Gain34 : Gain  Gain=w3TA
  Gain35 : Gain  Gain=w4HFL
  Gain36 : Gain  Gain=w5GLU
  Gain37 : Gain  Gain=w5HAM
  Gain38 : Gain  Gain=w5BFSH
  Gain39 : Gain  Gain=w5VAS
  Gain4 : Gain  Gain=w1VAS
  Gain40 : Gain  Gain=w5RF
  Gain41 : Gain  Gain=w5GAS
  Gain42 : Gain  Gain=w5SOL
  Gain43 : Gain  Gain=w5TA
  Gain44 : Gain  Gain=w5HFL
  Gain5 : Gain  Gain=w1RF
  Gain6 : Gain  Gain=w1GAS
  Gain7 : Gain  Gain=w1SOL
  Gain8 : Gain  Gain=w1TA
  Gain9 : Gain  Gain=w2HFL
  Less Than{,1..9} (10 alike) : RelationalOperator  Operator=<=  OutDataTypeStr=boolean  RndMeth=Simplest  InputSameDT=off
  Logical Operator{,1..4} (5 alike) : Logic  AllPortsSameDT=off  OutDataTypeStr=boolean
  Mux : Mux  Inputs=9
  Pulse 0 : Subsystem
  Pulse 1 : Subsystem
  Pulse 2 : Subsystem
  Pulse 3 : Subsystem
  Pulse 4 : Subsystem
  Sum{,2,4,6,8} (5 alike) : Sum  Inputs=|++
  Sum{1,3,5,7,9} (5 alike) : Sum  Inputs=|+-
  Sum{10..18} (9 alike) : Sum  Inputs=+++++
  Switch{,1..4} (5 alike) : Switch  Criteria=u2 > Threshold  SaturateOnIntegerOverflow=off  InputSameDT=off
  Zero{,1..4} (5 alike) : Constant  Value=0  OutDataTypeStr=Inherit: Inherit via back propagation
  Outport : Outport
  wires:
  Mux/1 -> Outport/1
  Sum18/1 -> Mux/9
  Sum17/1 -> Mux/8
  Sum16/1 -> Mux/7
  Sum15/1 -> Mux/6
  Sum14/1 -> Mux/5
  Sum13/1 -> Mux/4
  Sum12/1 -> Mux/3
  Sum11/1 -> Mux/2
  Sum10/1 -> Mux/1
  Gain4/1 -> Sum14/1
  Gain3/1 -> Sum15/1
  Gain6/1 -> Sum16/1
  Gain13/1 -> Sum14/2
  Gain12/1 -> Sum15/2
  Gain15/1 -> Sum16/2
  Gain29/1 -> Sum15/3
  Gain32/1 -> Sum16/3
  Gain22/1 -> Sum15/4
  Gain25/1 -> Sum16/4
  Gain41/1 -> Sum16/5
  Gain38/1 -> Sum15/5
  Gain39/1 -> Sum14/5
  Gain23/1 -> Sum14/4
  Gain30/1 -> Sum14/3
  Gain40/1 -> Sum13/5
  Gain24/1 -> Sum13/4
  Gain14/1 -> Sum13/2
  Gain5/1 -> Sum13/1
  Gain31/1 -> Sum13/3
  Gain37/1 -> Sum12/5
  Gain21/1 -> Sum12/4
  Gain28/1 -> Sum12/3
  Gain11/1 -> Sum12/2
  Gain2/1 -> Sum12/1
  Gain36/1 -> Sum11/5
  Gain20/1 -> Sum11/4
  Gain19/1 -> Sum11/3
  Gain10/1 -> Sum11/2
  Gain1/1 -> Sum11/1
  Gain7/1 -> Sum17/1
  Gain16/1 -> Sum17/2
  Gain33/1 -> Sum17/3
  Gain26/1 -> Sum17/4
  Gain42/1 -> Sum17/5
  Gain8/1 -> Sum18/1
  Gain17/1 -> Sum18/2
  Gain34/1 -> Sum18/3
  Gain27/1 -> Sum18/4
  Gain43/1 -> Sum18/5
  Gain44/1 -> Sum10/5
  Gain35/1 -> Sum10/4
  Gain18/1 -> Sum10/3
  Gain9/1 -> Sum10/2
  Gain/1 -> Sum10/1
  [Pulse5_4] -> Gain38/1, Gain43/1, Gain42/1, Gain41/1, Gain39/1, Gain40/1, Gain37/1, Gain36/1, Gain44/1
  [Pulse3_4] -> Gain29/1, Gain34/1, Gain33/1, Gain32/1, Gain30/1, Gain31/1, Gain28/1, Gain19/1, Gain18/1
  [Pulse4_4] -> Gain35/1, Gain20/1, Gain21/1, Gain24/1, Gain23/1, Gain25/1, Gain26/1, Gain27/1, Gain22/1
  [Pulse2_4] -> Gain12/1, Gain17/1, Gain16/1, Gain15/1, Gain13/1, Gain14/1, Gain11/1, Gain10/1, Gain9/1
  [Pulse1_4] -> Gain/1, Gain1/1, Gain2/1, Gain5/1, Gain4/1, Gain6/1, Gain7/1, Gain8/1, Gain3/1
  Inport/1 -> Less Than/2, Less Than1/1, Pulse 0/1(phi out), Less Than3/1, Less Than2/2, Pulse 1/1(phi out), Pulse 2/1(phi out), Less Than7/1, Less Than6/2, Pulse 3/1(phi out), Pulse 4/1(phi out), Less Than8/2, Less Than9/1, Less Than4/2, Less Than5/1
  Constant1/1 -> Sum/1, Sum1/1
  Constant9/1 -> Sum8/1, Sum9/1
  Less Than3/1 -> Logical Operator1/2
  Sum4/1 -> Less Than5/2
  Less Than9/1 -> Logical Operator4/2
  Sum7/1 -> Less Than6/1
  Sum2/1 -> Less Than3/2
  Zero1/1 -> Switch1/3
  Less Than8/1 -> Logical Operator4/1
  Constant2/1 -> Sum3/1, Sum2/1
  Logical Operator3/1 -> Switch3/2
  Less Than7/1 -> Logical Operator3/2
  Constant10/1 -> Sum8/2, Sum9/2
  Switch1/1 -> [Pulse2_4]
  Less Than6/1 -> Logical Operator3/1
  Less Than1/1 -> Logical Operator/2
  Sum8/1 -> Less Than9/2
  Zero/1 -> Switch/3
  Sum9/1 -> Less Than8/1
  Logical Operator4/1 -> Switch4/2
  Constant8/1 -> Sum7/2, Sum6/2
  Sum6/1 -> Less Than7/2
  Constant4/1 -> Sum3/2, Sum2/2
  Constant7/1 -> Sum7/1, Sum6/1
  Sum3/1 -> Less Than2/1
  Switch3/1 -> [Pulse4_4]
  Zero3/1 -> Switch3/3
  Switch/1 -> [Pulse1_4]
  Less Than2/1 -> Logical Operator1/1
  Sum5/1 -> Less Than4/1
  Pulse 3/1(Out1) -> Switch3/1
  Switch2/1 -> [Pulse3_4]
  Zero2/1 -> Switch2/3
  Sum1/1 -> Less Than/1
  Pulse 1/1(Out1) -> Switch1/1
  Logical Operator1/1 -> Switch1/2
  Logical Operator/1 -> Switch/2
  Switch4/1 -> [Pulse5_4]
  Zero4/1 -> Switch4/3
  Less Than/1 -> Logical Operator/1
  Constant3/1 -> Sum/2, Sum1/2
  Pulse 0/1(Out1) -> Switch/1
  Sum/1 -> Less Than1/2
  Less Than4/1 -> Logical Operator2/1
  Less Than5/1 -> Logical Operator2/2
  Constant5/1 -> Sum4/1, Sum5/1
  Constant6/1 -> Sum4/2, Sum5/2
  Logical Operator2/1 -> Switch2/2
  Pulse 4/1(Out1) -> Switch4/1
  Pulse 2/1(Out1) -> Switch2/1

== system nms_sim_2D_cost/CPG-reflex-synergy controller/Reflexes1/IN RC1 ==
  in : Inport
  Constant : Constant  Value=tau_act_diRusso
  Divide : Product  Inputs=*/
  Integrator : Integrator  InitialCondition=init_exc
  Sum : Sum  Inputs=+-|
  out : Outport  VectorParamsAs1DForOutWhenUnconnected=off
  wires:
  Constant/1 -> Divide/2
  in/1 -> Sum/1
  Integrator/1 -> out/1, Sum/2  "A"
  Divide/1 -> Integrator/1  "dA"
  Sum/1 -> Divide/1

== system nms_sim_2D_cost/CPG-reflex-synergy controller/Reflexes1/IN RC10 ==
  in : Inport
  Constant : Constant  Value=tau_act_diRusso
  Divide : Product  Inputs=*/
  Integrator : Integrator  InitialCondition=init_exc
  Sum : Sum  Inputs=+-|
  out : Outport  VectorParamsAs1DForOutWhenUnconnected=off
  wires:
  Constant/1 -> Divide/2
  in/1 -> Sum/1
  Integrator/1 -> out/1, Sum/2  "A"
  Divide/1 -> Integrator/1  "dA"
  Sum/1 -> Divide/1

== system nms_sim_2D_cost/CPG-reflex-synergy controller/Reflexes1/IN RC11 ==
  in : Inport
  Constant : Constant  Value=tau_act_diRusso
  Divide : Product  Inputs=*/
  Integrator : Integrator  InitialCondition=init_exc
  Sum : Sum  Inputs=+-|
  out : Outport  VectorParamsAs1DForOutWhenUnconnected=off
  wires:
  Constant/1 -> Divide/2
  in/1 -> Sum/1
  Integrator/1 -> out/1, Sum/2  "A"
  Divide/1 -> Integrator/1  "dA"
  Sum/1 -> Divide/1

== system nms_sim_2D_cost/CPG-reflex-synergy controller/Reflexes1/IN RC12 ==
  in : Inport
  Constant : Constant  Value=tau_act_diRusso
  Divide : Product  Inputs=*/
  Integrator : Integrator  InitialCondition=init_exc
  Sum : Sum  Inputs=+-|
  out : Outport  VectorParamsAs1DForOutWhenUnconnected=off
  wires:
  Constant/1 -> Divide/2
  in/1 -> Sum/1
  Integrator/1 -> out/1, Sum/2  "A"
  Divide/1 -> Integrator/1  "dA"
  Sum/1 -> Divide/1

== system nms_sim_2D_cost/CPG-reflex-synergy controller/Reflexes1/IN RC13 ==
  in : Inport
  Constant : Constant  Value=tau_act_diRusso
  Divide : Product  Inputs=*/
  Integrator : Integrator  InitialCondition=init_exc
  Sum : Sum  Inputs=+-|
  out : Outport  VectorParamsAs1DForOutWhenUnconnected=off
  wires:
  Constant/1 -> Divide/2
  in/1 -> Sum/1
  Integrator/1 -> out/1, Sum/2  "A"
  Divide/1 -> Integrator/1  "dA"
  Sum/1 -> Divide/1

== system nms_sim_2D_cost/CPG-reflex-synergy controller/Reflexes1/IN RC14 ==
  in : Inport
  Constant : Constant  Value=tau_act_diRusso
  Divide : Product  Inputs=*/
  Integrator : Integrator  InitialCondition=init_exc
  Sum : Sum  Inputs=+-|
  out : Outport  VectorParamsAs1DForOutWhenUnconnected=off
  wires:
  Constant/1 -> Divide/2
  in/1 -> Sum/1
  Integrator/1 -> out/1, Sum/2  "A"
  Divide/1 -> Integrator/1  "dA"
  Sum/1 -> Divide/1

== system nms_sim_2D_cost/CPG-reflex-synergy controller/Reflexes1/IN RC15 ==
  in : Inport
  Constant : Constant  Value=tau_act_diRusso
  Divide : Product  Inputs=*/
  Integrator : Integrator  InitialCondition=init_exc
  Sum : Sum  Inputs=+-|
  out : Outport  VectorParamsAs1DForOutWhenUnconnected=off
  wires:
  Constant/1 -> Divide/2
  in/1 -> Sum/1
  Integrator/1 -> out/1, Sum/2  "A"
  Divide/1 -> Integrator/1  "dA"
  Sum/1 -> Divide/1

== system nms_sim_2D_cost/CPG-reflex-synergy controller/Reflexes1/IN RC16 ==
  in : Inport
  Constant : Constant  Value=tau_act_diRusso
  Divide : Product  Inputs=*/
  Integrator : Integrator  InitialCondition=init_exc
  Sum : Sum  Inputs=+-|
  out : Outport  VectorParamsAs1DForOutWhenUnconnected=off
  wires:
  Constant/1 -> Divide/2
  in/1 -> Sum/1
  Integrator/1 -> out/1, Sum/2  "A"
  Divide/1 -> Integrator/1  "dA"
  Sum/1 -> Divide/1

== system nms_sim_2D_cost/CPG-reflex-synergy controller/Reflexes1/IN RC17 ==
  in : Inport
  Constant : Constant  Value=tau_act_diRusso
  Divide : Product  Inputs=*/
  Integrator : Integrator  InitialCondition=init_exc
  Sum : Sum  Inputs=+-|
  out : Outport  VectorParamsAs1DForOutWhenUnconnected=off
  wires:
  Constant/1 -> Divide/2
  in/1 -> Sum/1
  Integrator/1 -> out/1, Sum/2  "A"
  Divide/1 -> Integrator/1  "dA"
  Sum/1 -> Divide/1

== system nms_sim_2D_cost/CPG-reflex-synergy controller/Reflexes1/IN RC18 ==
  in : Inport
  Constant : Constant  Value=tau_act_diRusso
  Divide : Product  Inputs=*/
  Integrator : Integrator  InitialCondition=init_exc
  Sum : Sum  Inputs=+-|
  out : Outport  VectorParamsAs1DForOutWhenUnconnected=off
  wires:
  Constant/1 -> Divide/2
  in/1 -> Sum/1
  Integrator/1 -> out/1, Sum/2  "A"
  Divide/1 -> Integrator/1  "dA"
  Sum/1 -> Divide/1

== system nms_sim_2D_cost/CPG-reflex-synergy controller/Reflexes1/IN RC19 ==
  in : Inport
  Constant : Constant  Value=tau_act_diRusso
  Divide : Product  Inputs=*/
  Integrator : Integrator  InitialCondition=init_exc
  Sum : Sum  Inputs=+-|
  out : Outport  VectorParamsAs1DForOutWhenUnconnected=off
  wires:
  Constant/1 -> Divide/2
  in/1 -> Sum/1
  Integrator/1 -> out/1, Sum/2  "A"
  Divide/1 -> Integrator/1  "dA"
  Sum/1 -> Divide/1

== system nms_sim_2D_cost/CPG-reflex-synergy controller/Reflexes1/IN RC2 ==
  in : Inport
  Constant : Constant  Value=tau_act_diRusso
  Divide : Product  Inputs=*/
  Integrator : Integrator  InitialCondition=init_exc
  Sum : Sum  Inputs=+-|
  out : Outport  VectorParamsAs1DForOutWhenUnconnected=off
  wires:
  Constant/1 -> Divide/2
  in/1 -> Sum/1
  Integrator/1 -> out/1, Sum/2  "A"
  Divide/1 -> Integrator/1  "dA"
  Sum/1 -> Divide/1

== system nms_sim_2D_cost/CPG-reflex-synergy controller/Reflexes1/IN RC20 ==
  in : Inport
  Constant : Constant  Value=tau_act_diRusso
  Divide : Product  Inputs=*/
  Integrator : Integrator  InitialCondition=init_exc
  Sum : Sum  Inputs=+-|
  out : Outport  VectorParamsAs1DForOutWhenUnconnected=off
  wires:
  Constant/1 -> Divide/2
  in/1 -> Sum/1
  Integrator/1 -> out/1, Sum/2  "A"
  Divide/1 -> Integrator/1  "dA"
  Sum/1 -> Divide/1

== system nms_sim_2D_cost/CPG-reflex-synergy controller/Reflexes1/IN RC21 ==
  in : Inport
  Constant : Constant  Value=tau_act_diRusso
  Divide : Product  Inputs=*/
  Integrator : Integrator  InitialCondition=init_exc
  Sum : Sum  Inputs=+-|
  out : Outport  VectorParamsAs1DForOutWhenUnconnected=off
  wires:
  Constant/1 -> Divide/2
  in/1 -> Sum/1
  Integrator/1 -> out/1, Sum/2  "A"
  Divide/1 -> Integrator/1  "dA"
  Sum/1 -> Divide/1

== system nms_sim_2D_cost/CPG-reflex-synergy controller/Reflexes1/IN RC22 ==
  in : Inport
  Constant : Constant  Value=tau_act_diRusso
  Divide : Product  Inputs=*/
  Integrator : Integrator  InitialCondition=init_exc
  Sum : Sum  Inputs=+-|
  out : Outport  VectorParamsAs1DForOutWhenUnconnected=off
  wires:
  Constant/1 -> Divide/2
  in/1 -> Sum/1
  Integrator/1 -> out/1, Sum/2  "A"
  Divide/1 -> Integrator/1  "dA"
  Sum/1 -> Divide/1

== system nms_sim_2D_cost/CPG-reflex-synergy controller/Reflexes1/IN RC23 ==
  in : Inport
  Constant : Constant  Value=tau_act_diRusso
  Divide : Product  Inputs=*/
  Integrator : Integrator  InitialCondition=init_exc
  Sum : Sum  Inputs=+-|
  out : Outport  VectorParamsAs1DForOutWhenUnconnected=off
  wires:
  Constant/1 -> Divide/2
  in/1 -> Sum/1
  Integrator/1 -> out/1, Sum/2  "A"
  Divide/1 -> Integrator/1  "dA"
  Sum/1 -> Divide/1

== system nms_sim_2D_cost/CPG-reflex-synergy controller/Reflexes1/IN RC24 ==
  in : Inport
  Constant : Constant  Value=tau_act_diRusso
  Divide : Product  Inputs=*/
  Integrator : Integrator  InitialCondition=init_exc
  Sum : Sum  Inputs=+-|
  out : Outport  VectorParamsAs1DForOutWhenUnconnected=off
  wires:
  Constant/1 -> Divide/2
  in/1 -> Sum/1
  Integrator/1 -> out/1, Sum/2  "A"
  Divide/1 -> Integrator/1  "dA"
  Sum/1 -> Divide/1
